simulink model "ex8"  (Simulink 7.6)
settings: Solver=FixedStepDiscrete  SolverMode=SingleTasking  StartTime=0.0  StopTime=10.0  FixedStep=0.001  RelTol=1e-3
libraries: simulink x12, dsPICdrivers x9
settings Model: Creator=Lior  LastModifiedBy=Lior  BufferReuse=off
settings OptimizationCC: BlockReduction=off  InlineParams=on  BufferReuse=off  OptimizeModelRefInitCode=on  LifeSpan=1
settings HardwareCC: ProdBitPerInt=16  ProdBitPerPointer=16  ProdEndianess=LittleEndian  ProdWordSize=16  ProdHWDeviceType=16-bit Generic
settings RTWCC: SystemTargetFile=dspic.tlc  MakeCommand=make_CreateMPLAB  TemplateMakefile=dspic_pic30_gcc.tmf  PostCodeGenCommand=dsPIC_Compile()  Description=Embedded Target for Microchip dsPIC (real-time)  ProcessScript=dspic_make_rtw_hook
settings CodeAppCC: IgnoreCustomStorageClasses=off
settings STFCustomTargetCC: IncludeMdlTerminateFcn=off  CombineOutputUpdateFcns=on  SuppressErrorStatus=on  ERTCustomFileBanners=on  SupportContinuousTime=off  SupportNonInlinedSFcns=off  SystemTargetFile=dspic.tlc
settings ERTTargetCC: MultiwordLength=2048  ParMdlRefBuildCompliant=off  CompOptLevelCompliant=off  IncludeMdlTerminateFcn=off  SuppressErrorStatus=on  ERTFirstTimeCompliant=off  ModelStepFunctionPrototypeControlCompliant=off  CPPClassGenCompliant=off  ExtModeMexFile=ext_serial_win32_comm  InlinedParameterPlacement=NonHierarchical  ERTSrcFileBannerTemplate=dsPIC_code_template.cgt  ERTHdrFileBannerTemplate=dsPIC_code_template.cgt  ERTDataSrcFileTemplate=dsPIC_code_template.cgt  ERTDataHdrFileTemplate=dsPIC_code_template.cgt  ERTCustomFileTemplate=dsPIC_main.tlc  ConvertIfToSwitch=off
settings CustomProperty: DataType=string  Value=C:\PROGRA~1\MATLAB\R2010b\bin\win64\gmake

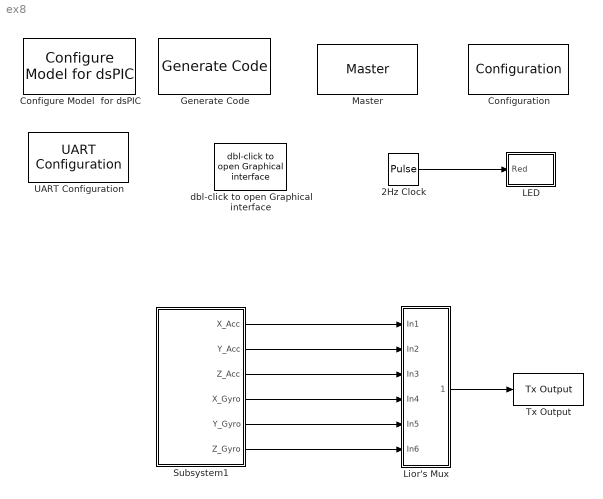
== system ex8 ==
  2Hz Clock : DiscretePulseGenerator  PulseType=Time based  Period=0.2  PulseWidth=50
  Configuration : dsPICdrivers/Configuration  SystemSampleTime=-1  double64=off
  Configure Model  for dsPIC : dsPICdrivers/Simulink Configuration/Configure Model  for dsPIC
  Generate Code : dsPICdrivers/Simulink Configuration/Generate Code
  LED : Subsystem
  Lior's Mux : Subsystem
  Master : dsPICdrivers/Master  Tag=dsPIC_MASTER  Priority=1  TimeStepType=Timer1  picType=33fJ256MC710  fcy=7500000  Quartz_33f=15e6  PLLActive_33f=off  fcyDesired_33f=0  tmr1="[1  7499  0]"  tmr1Info="Time Step : 0.001  ;   Error : 0%  PR1=7499"  tmr2345="[0  0  0  0  0  0  0  0]"  tmr2345cfg=[-1 -1 -1 -1 -1 -1 -1 -1]  IOautoConf=on  typePort="[ 0   0   0   0   0   0   0   0   0   0   0   0   0   0   0   0   8   8   0   0   8   8   8   8   0   0   0   0   0   0   0   0   0   0   0   0   0   0   0   0   0   0   0   0   0   0   0   0   0   0   0   0   0   0   0   0   0   0   0   0   0   0   0   0   0   0   0   0  10   0   0   0   0   0   0   0   0   0   0   0   0   0   4   5   0   0   0   0   0   0   0   0   0   0   0   0   0   0   0   0   0   0   0   0   0   0   0   0   0   0   0   0 ]"  TRIS="[ 65535  65535  65535  65535  65519  65535  65535 ]"  ADPCFG=0  MasterBusyPort=None  MasterOverloadPort=None  FOSC=Quartz (XT - HS)  ClockSwitchMonitor=Both disabled  TempProtection_33f=TEMP_ON  FPBOR=<empty>  PWRT=disable  MCLR=<empty>  ICD=ICS_PGD1  JTAGEN=JTAGEN_OFF  PowerSave=off  OverrideFcy=off  NewFcy=1e6  PR2345="[65535  65535  65535  65535  65535  65535  65535  65535]"
  Subsystem1 : Subsystem
  Tx Output : dsPICdrivers/Serial PORT/Tx Output  Tag=dsPIC_TX  Priority=5  UART=1  OrderingInOutPopup=None
  UART Configuration : dsPICdrivers/Serial PORT/UART Configuration  Tag=dsPIC_config_UART  Priority=2  UART=1  proposed_BAUD=115200  BAUD=115200  ALT_TX_RX=on  InterruptTxWhen=When Transmit Buffer is empty  TXInterruptPri=1  TxBufferSize=32  TXEN=on  InterruptRxWhen=When Receive Buffer is full (contain 4 characters)  RXInterruptPri=2  RxBufferSize=32  DoNotImplementRxInterrupt=off  DoNotImplementTxInterrupt=off  UxBRG=3  Info="UxBRG = 3   ||  Real Baud : 117188   ||  % error : 1.7253  ||  max 11.7188 Bytes / Step"  RealBaud=0  ERROR=1.7253  BYTES_STEP=11.7188
  dbl-click to open Graphical interface : dsPICdrivers/Serial PORT/dbl-click to open Graphical interface  Nothing=0
  wires:
  2Hz Clock/1 -> LED/1(Red)
  Lior's Mux/1(Out1) -> Tx Output/1
  Subsystem1/1(X_Acc) -> Lior's Mux/1(In1)
  Subsystem1/2(Y_Acc) -> Lior's Mux/2(In2)
  Subsystem1/3(Z_Acc) -> Lior's Mux/3(In3)
  Subsystem1/4(X_Gyro) -> Lior's Mux/4(In4)
  Subsystem1/5(Y_Gyro) -> Lior's Mux/5(In5)
  Subsystem1/6(Z_Gyro) -> Lior's Mux/6(In6)

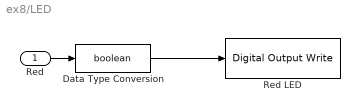
== system ex8/LED ==
  Red : Inport
  Data Type Conversion : DataTypeConversion  OutDataTypeStr=boolean
  Red LED : dsPICdrivers/Digital I//O/Digital Output Write  Tag=dsPIC_Digital_Output  Priority=5  PORT=E  Pin=[4]  Simultaneous=off  OrderingInOutPopup=None
  wires:
  Data Type Conversion/1 -> Red LED/1
  Red/1 -> Data Type Conversion/1

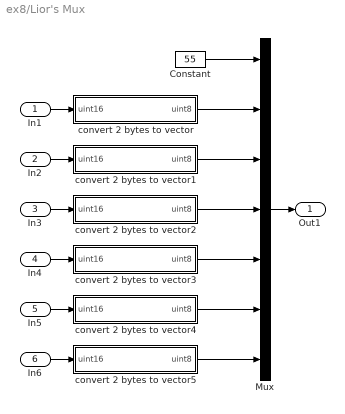
== system ex8/Lior's Mux ==
  In1 : Inport
  In2 : Inport  Port=2
  In3 : Inport  Port=3
  In4 : Inport  Port=4
  In5 : Inport  Port=5
  In6 : Inport  Port=6
  Constant : Constant  Value=55  OutDataTypeStr=uint8  SampleTime=0.01
  Mux : Mux  Inputs=7
  convert 2 bytes to vector : Subsystem
  convert 2 bytes to vector1 : Subsystem
  convert 2 bytes to vector2 : Subsystem
  convert 2 bytes to vector3 : Subsystem
  convert 2 bytes to vector4 : Subsystem
  convert 2 bytes to vector5 : Subsystem
  Out1 : Outport
  wires:
  In1/1 -> convert 2 bytes to vector/1(uint16)
  In2/1 -> convert 2 bytes to vector1/1(uint16)
  In3/1 -> convert 2 bytes to vector2/1(uint16)
  Mux/1 -> Out1/1
  In4/1 -> convert 2 bytes to vector3/1(uint16)
  In5/1 -> convert 2 bytes to vector4/1(uint16)
  In6/1 -> convert 2 bytes to vector5/1(uint16)
  Constant/1 -> Mux/1
  convert 2 bytes to vector/1("uint8 ") -> Mux/2
  convert 2 bytes to vector1/1("uint8 ") -> Mux/3
  convert 2 bytes to vector2/1("uint8 ") -> Mux/4
  convert 2 bytes to vector3/1("uint8 ") -> Mux/5
  convert 2 bytes to vector4/1("uint8 ") -> Mux/6
  convert 2 bytes to vector5/1("uint8 ") -> Mux/7

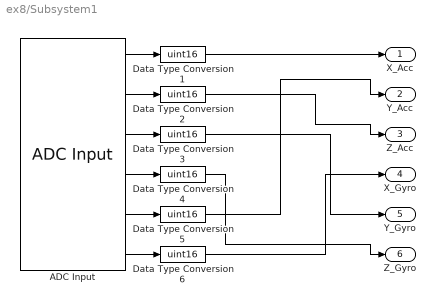
== system ex8/Subsystem1 ==
  ADC Input : dsPICdrivers/Peripheral I//O/ADC Input  Tag=dsPIC_ADC  Priority=5  ADC_TYPE=12 bits  ADC_MODE=Continuous sampling & get last channel value  NbrSampleStep=1  VoltRefpopup="AVdd  -  AVss"  OutFormatBitspopup=0000 dddd dddd dddd : Integer  InterruptPriority=6  ANCHANNELS=[0 6 1 7 4 5]  MaxName=ANmax = 4095  Rin=1e2  ADCS=9  SAMC=1  Temperature=25  DMAChannel=4  SampleTime=0.004  Status="OK  |  Tsmp=6.667e-007 |  T/Channel=1.000e-005 |  Tall=6.000e-005"  SSRC=auto convert
  Data Type Conversion{1..6} (6 alike) : DataTypeConversion  OutDataTypeStr=uint16
  X_Acc : Outport
  Y_Acc : Outport  Port=2
  Z_Acc : Outport  Port=3
  X_Gyro : Outport  Port=4
  Y_Gyro : Outport  Port=5
  Z_Gyro : Outport  Port=6
  wires:
  ADC Input/1 -> Data Type Conversion1/1
  ADC Input/2 -> Data Type Conversion2/1
  ADC Input/3 -> Data Type Conversion3/1
  ADC Input/4 -> Data Type Conversion4/1
  ADC Input/5 -> Data Type Conversion5/1
  ADC Input/6 -> Data Type Conversion6/1
  Data Type Conversion1/1 -> X_Acc/1
  Data Type Conversion2/1 -> Z_Acc/1
  Data Type Conversion3/1 -> Y_Gyro/1
  Data Type Conversion4/1 -> Z_Gyro/1
  Data Type Conversion5/1 -> Y_Acc/1
  Data Type Conversion6/1 -> X_Gyro/1

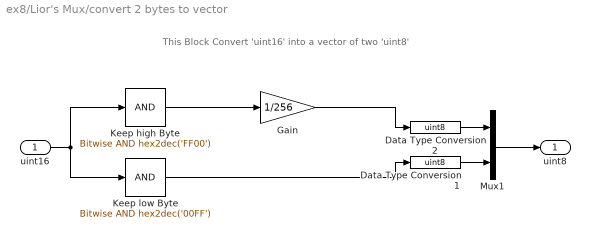
== system ex8/Lior's Mux/convert 2 bytes to vector ==
  note: This Block Convert 'uint16' into a vector of two 'uint8'
  uint16 : Inport
  Data Type Conversion1 : DataTypeConversion  OutDataTypeStr=uint8
  Data Type Conversion2 : DataTypeConversion  OutDataTypeStr=uint8
  Gain : Gain  Gain=1/256  OutDataTypeStr=uint8
  Keep high Byte : simulink/Logic and Bit Operations/Bitwise Operator  logicop=AND  UseBitMask=on  BitMask=hex2dec('FF00')  BitMaskRealWorld=Stored Integer
  Keep low Byte : simulink/Logic and Bit Operations/Bitwise Operator  logicop=AND  UseBitMask=on  BitMask=hex2dec('00FF')  BitMaskRealWorld=Stored Integer
  Mux1 : Mux  Inputs=2
  "uint8 " : Outport
  wires:
  uint16/1 -> Keep low Byte/1, Keep high Byte/1
  Keep high Byte/1 -> Gain/1
  Gain/1 -> Data Type Conversion2/1
  Keep low Byte/1 -> Data Type Conversion1/1
  Data Type Conversion2/1 -> Mux1/1
  Data Type Conversion1/1 -> Mux1/2
  Mux1/1 -> "uint8 "/1

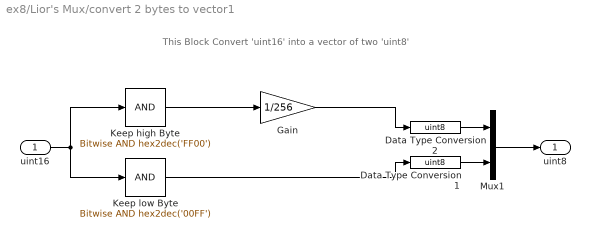
== system ex8/Lior's Mux/convert 2 bytes to vector1 ==
  note: This Block Convert 'uint16' into a vector of two 'uint8'
  uint16 : Inport
  Data Type Conversion1 : DataTypeConversion  OutDataTypeStr=uint8
  Data Type Conversion2 : DataTypeConversion  OutDataTypeStr=uint8
  Gain : Gain  Gain=1/256  OutDataTypeStr=uint8
  Keep high Byte : simulink/Logic and Bit Operations/Bitwise Operator  logicop=AND  UseBitMask=on  BitMask=hex2dec('FF00')  BitMaskRealWorld=Stored Integer
  Keep low Byte : simulink/Logic and Bit Operations/Bitwise Operator  logicop=AND  UseBitMask=on  BitMask=hex2dec('00FF')  BitMaskRealWorld=Stored Integer
  Mux1 : Mux  Inputs=2
  "uint8 " : Outport
  wires:
  Mux1/1 -> "uint8 "/1
  Data Type Conversion1/1 -> Mux1/2
  Data Type Conversion2/1 -> Mux1/1
  Keep low Byte/1 -> Data Type Conversion1/1
  Gain/1 -> Data Type Conversion2/1
  Keep high Byte/1 -> Gain/1
  uint16/1 -> Keep high Byte/1, Keep low Byte/1

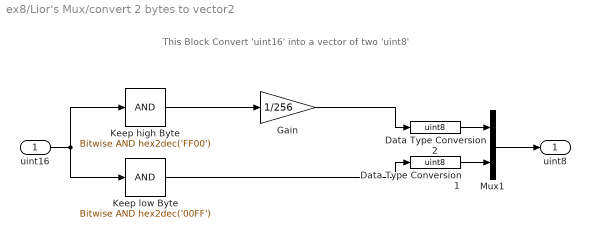
== system ex8/Lior's Mux/convert 2 bytes to vector2 ==
  note: This Block Convert 'uint16' into a vector of two 'uint8'
  uint16 : Inport
  Data Type Conversion1 : DataTypeConversion  OutDataTypeStr=uint8
  Data Type Conversion2 : DataTypeConversion  OutDataTypeStr=uint8
  Gain : Gain  Gain=1/256  OutDataTypeStr=uint8
  Keep high Byte : simulink/Logic and Bit Operations/Bitwise Operator  logicop=AND  UseBitMask=on  BitMask=hex2dec('FF00')  BitMaskRealWorld=Stored Integer
  Keep low Byte : simulink/Logic and Bit Operations/Bitwise Operator  logicop=AND  UseBitMask=on  BitMask=hex2dec('00FF')  BitMaskRealWorld=Stored Integer
  Mux1 : Mux  Inputs=2
  "uint8 " : Outport
  wires:
  uint16/1 -> Keep low Byte/1, Keep high Byte/1
  Keep high Byte/1 -> Gain/1
  Gain/1 -> Data Type Conversion2/1
  Keep low Byte/1 -> Data Type Conversion1/1
  Data Type Conversion2/1 -> Mux1/1
  Data Type Conversion1/1 -> Mux1/2
  Mux1/1 -> "uint8 "/1

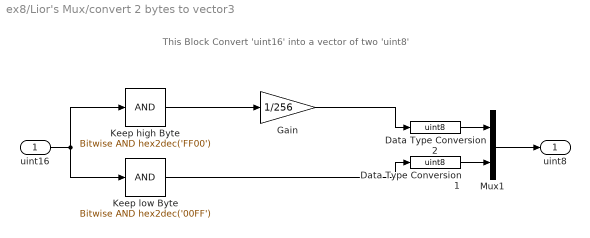
== system ex8/Lior's Mux/convert 2 bytes to vector3 ==
  note: This Block Convert 'uint16' into a vector of two 'uint8'
  uint16 : Inport
  Data Type Conversion1 : DataTypeConversion  OutDataTypeStr=uint8
  Data Type Conversion2 : DataTypeConversion  OutDataTypeStr=uint8
  Gain : Gain  Gain=1/256  OutDataTypeStr=uint8
  Keep high Byte : simulink/Logic and Bit Operations/Bitwise Operator  logicop=AND  UseBitMask=on  BitMask=hex2dec('FF00')  BitMaskRealWorld=Stored Integer
  Keep low Byte : simulink/Logic and Bit Operations/Bitwise Operator  logicop=AND  UseBitMask=on  BitMask=hex2dec('00FF')  BitMaskRealWorld=Stored Integer
  Mux1 : Mux  Inputs=2
  "uint8 " : Outport
  wires:
  Mux1/1 -> "uint8 "/1
  Data Type Conversion1/1 -> Mux1/2
  Data Type Conversion2/1 -> Mux1/1
  Keep low Byte/1 -> Data Type Conversion1/1
  Gain/1 -> Data Type Conversion2/1
  Keep high Byte/1 -> Gain/1
  uint16/1 -> Keep high Byte/1, Keep low Byte/1

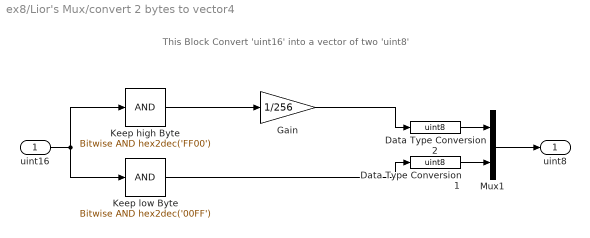
== system ex8/Lior's Mux/convert 2 bytes to vector4 ==
  note: This Block Convert 'uint16' into a vector of two 'uint8'
  uint16 : Inport
  Data Type Conversion1 : DataTypeConversion  OutDataTypeStr=uint8
  Data Type Conversion2 : DataTypeConversion  OutDataTypeStr=uint8
  Gain : Gain  Gain=1/256  OutDataTypeStr=uint8
  Keep high Byte : simulink/Logic and Bit Operations/Bitwise Operator  logicop=AND  UseBitMask=on  BitMask=hex2dec('FF00')  BitMaskRealWorld=Stored Integer
  Keep low Byte : simulink/Logic and Bit Operations/Bitwise Operator  logicop=AND  UseBitMask=on  BitMask=hex2dec('00FF')  BitMaskRealWorld=Stored Integer
  Mux1 : Mux  Inputs=2
  "uint8 " : Outport
  wires:
  uint16/1 -> Keep low Byte/1, Keep high Byte/1
  Keep high Byte/1 -> Gain/1
  Gain/1 -> Data Type Conversion2/1
  Keep low Byte/1 -> Data Type Conversion1/1
  Data Type Conversion2/1 -> Mux1/1
  Data Type Conversion1/1 -> Mux1/2
  Mux1/1 -> "uint8 "/1

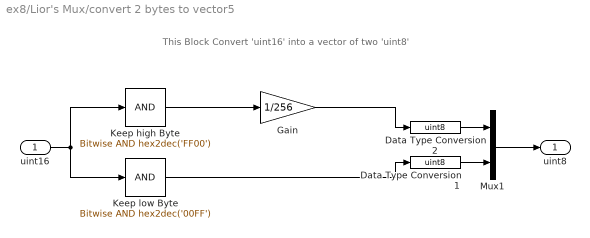
== system ex8/Lior's Mux/convert 2 bytes to vector5 ==
  note: This Block Convert 'uint16' into a vector of two 'uint8'
  uint16 : Inport
  Data Type Conversion1 : DataTypeConversion  OutDataTypeStr=uint8
  Data Type Conversion2 : DataTypeConversion  OutDataTypeStr=uint8
  Gain : Gain  Gain=1/256  OutDataTypeStr=uint8
  Keep high Byte : simulink/Logic and Bit Operations/Bitwise Operator  logicop=AND  UseBitMask=on  BitMask=hex2dec('FF00')  BitMaskRealWorld=Stored Integer
  Keep low Byte : simulink/Logic and Bit Operations/Bitwise Operator  logicop=AND  UseBitMask=on  BitMask=hex2dec('00FF')  BitMaskRealWorld=Stored Integer
  Mux1 : Mux  Inputs=2
  "uint8 " : Outport
  wires:
  Mux1/1 -> "uint8 "/1
  Data Type Conversion1/1 -> Mux1/2
  Data Type Conversion2/1 -> Mux1/1
  Keep low Byte/1 -> Data Type Conversion1/1
  Gain/1 -> Data Type Conversion2/1
  Keep high Byte/1 -> Gain/1
  uint16/1 -> Keep high Byte/1, Keep low Byte/1
